simulink library "Spring_Control_None"  (R2025a)
settings: Solver=VariableStepAuto  StartTime=0.0  StopTime=10.0  RelTol=1e-3
Description:
  | Copyright 2026 The MathWorks, Inc.
settings Model: Creator=smiller  LastModifiedBy=smiller
settings OptimizationCC: ReuseModelBlockBuffer=off
settings ModelReferenceCC: EnableRefExpFcnMdlSchedulingChecks=on
settings RTWCC: GPUComputeCapability=3.5

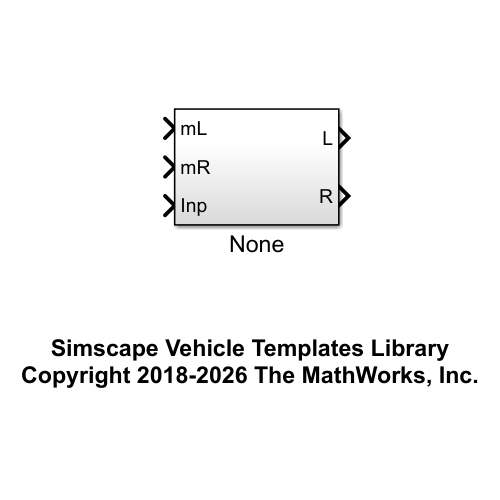
[thumbnail: Simulink's stored preview of the top-level diagram]
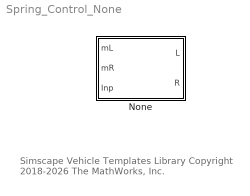
== system Spring_Control_None ==
  note: Simscape Vehicle Templates Library
      | Copyright 2018-2026 The MathWorks, Inc.
  None : Subsystem  VariantControl=Choice

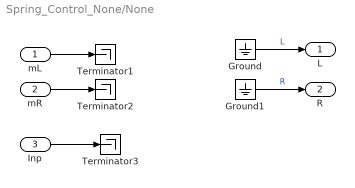
== system Spring_Control_None/None ==
  mL : Inport
  mR : Inport  Port=2
  Inp : Inport  Port=3
  Ground : Ground
  Ground1 : Ground
  Terminator1 : Terminator
  Terminator2 : Terminator
  Terminator3 : Terminator
  L : Outport  VectorParamsAs1DForOutWhenUnconnected=off
  R : Outport  Port=2  VectorParamsAs1DForOutWhenUnconnected=off
  wires:
  mR/1 -> Terminator2/1
  mL/1 -> Terminator1/1
  Ground1/1 -> R/1  "R"
  Ground/1 -> L/1  "L"
  Inp/1 -> Terminator3/1
